simulink model "kay1024_recursive_demo"  (R2021b)
settings: Solver=FixedStepDiscrete  StartTime=0.0  StopTime=420  FixedStep=1  RelTol=1e-3
InitFcn:
  | kay_demo_init;
undefined symbols (not defined in the file or in its folder): i
libraries: hdlBasic x1189, dspsrcs4 x16, vmcUtilities x1
(part 4 of 14)

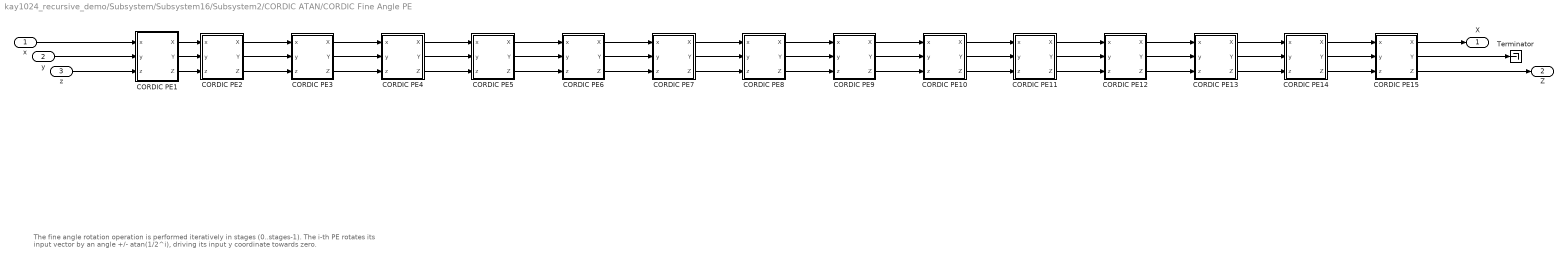
== system kay1024_recursive_demo/Subsystem/Subsystem16/Subsystem2/CORDIC ATAN/CORDIC Fine Angle PE ==
  note: The fine angle rotation operation is performed iteratively in stages (0..stages-1).
      | The i-th PE rotates its input vector by an angle +/- atan(1/2^i), driving its input y coordinate towards zero.
  x : Inport
  y : Inport  Port=2
  z : Inport  Port=3
  CORDIC PE1 : Subsystem  mask(CORDIC iteration PE){ii=0, pe_nbits=pe_nbits, pe_binpt=pe_binpt, epsilon_k_fcn=atan, epsilon_k=, pipeline=pipeline(1,1)}
      mask prompts: ii "Iteration Index ii"; pe_nbits "Number of X,Y,Z Bits"; pe_binpt "X,Y,Z Binary Point Position"; epsilon_k_fcn "Epsilon_k Function"; pipeline "Pipeline Latency"
      mask init: same as kay1024_recursive_demo/Subsystem/Subsystem16/Subsystem/CORDIC ATAN/CORDIC Fine Angle PE/CORDIC PE1
      mask TypeOptions epsilon_k_fcn: atan | atanh
      mask Display:
      | patch([0 iWidth iWidth 0],[0 0 iHeight iHeight] , bg);
      | patch(logoX,logoY , fg);
      | port_label('input',1,'x');
      | port_label('input',2,'y');
      | port_label('input',3,'z');
      | port_label('output',1,'X');
      | port_label('output',2,'Y');
      | port_label('output',3,'Z');
      | plot([0 0 iWidth iWidth 0], [0 iHeight iHeight 0 0]);
  CORDIC PE10 : Subsystem  mask(CORDIC iteration PE){ii=9, pe_nbits=pe_nbits, pe_binpt=pe_binpt, epsilon_k_fcn=atan, epsilon_k=, pipeline=pipeline(1,10)}
      mask prompts: ii "Iteration Index ii"; pe_nbits "Number of X,Y,Z Bits"; pe_binpt "X,Y,Z Binary Point Position"; epsilon_k_fcn "Epsilon_k Function"; pipeline "Pipeline Latency"
      mask init: same as kay1024_recursive_demo/Subsystem/Subsystem16/Subsystem/CORDIC ATAN/CORDIC Fine Angle PE/CORDIC PE1
      mask TypeOptions epsilon_k_fcn: atan | atanh
      mask Display:
      | patch([0 iWidth iWidth 0],[0 0 iHeight iHeight] , bg);
      | patch(logoX,logoY , fg);
      | port_label('input',1,'x');
      | port_label('input',2,'y');
      | port_label('input',3,'z');
      | port_label('output',1,'X');
      | port_label('output',2,'Y');
      | port_label('output',3,'Z');
      | plot([0 0 iWidth iWidth 0], [0 iHeight iHeight 0 0]);
  CORDIC PE11 : Subsystem  mask(CORDIC iteration PE){ii=10, pe_nbits=pe_nbits, pe_binpt=pe_binpt, epsilon_k_fcn=atan, epsilon_k=, pipeline=pipeline(1,11)}
      mask prompts: ii "Iteration Index ii"; pe_nbits "Number of X,Y,Z Bits"; pe_binpt "X,Y,Z Binary Point Position"; epsilon_k_fcn "Epsilon_k Function"; pipeline "Pipeline Latency"
      mask init: same as kay1024_recursive_demo/Subsystem/Subsystem16/Subsystem/CORDIC ATAN/CORDIC Fine Angle PE/CORDIC PE1
      mask TypeOptions epsilon_k_fcn: atan | atanh
      mask Display:
      | patch([0 iWidth iWidth 0],[0 0 iHeight iHeight] , bg);
      | patch(logoX,logoY , fg);
      | port_label('input',1,'x');
      | port_label('input',2,'y');
      | port_label('input',3,'z');
      | port_label('output',1,'X');
      | port_label('output',2,'Y');
      | port_label('output',3,'Z');
      | plot([0 0 iWidth iWidth 0], [0 iHeight iHeight 0 0]);
  CORDIC PE12 : Subsystem  mask(CORDIC iteration PE){ii=11, pe_nbits=pe_nbits, pe_binpt=pe_binpt, epsilon_k_fcn=atan, epsilon_k=, pipeline=pipeline(1,12)}
      mask prompts: ii "Iteration Index ii"; pe_nbits "Number of X,Y,Z Bits"; pe_binpt "X,Y,Z Binary Point Position"; epsilon_k_fcn "Epsilon_k Function"; pipeline "Pipeline Latency"
      mask init: same as kay1024_recursive_demo/Subsystem/Subsystem16/Subsystem/CORDIC ATAN/CORDIC Fine Angle PE/CORDIC PE1
      mask TypeOptions epsilon_k_fcn: atan | atanh
      mask Display:
      | patch([0 iWidth iWidth 0],[0 0 iHeight iHeight] , bg);
      | patch(logoX,logoY , fg);
      | port_label('input',1,'x');
      | port_label('input',2,'y');
      | port_label('input',3,'z');
      | port_label('output',1,'X');
      | port_label('output',2,'Y');
      | port_label('output',3,'Z');
      | plot([0 0 iWidth iWidth 0], [0 iHeight iHeight 0 0]);
  CORDIC PE13 : Subsystem  mask(CORDIC iteration PE){ii=12, pe_nbits=pe_nbits, pe_binpt=pe_binpt, epsilon_k_fcn=atan, epsilon_k=, pipeline=pipeline(1,13)}
      mask prompts: ii "Iteration Index ii"; pe_nbits "Number of X,Y,Z Bits"; pe_binpt "X,Y,Z Binary Point Position"; epsilon_k_fcn "Epsilon_k Function"; pipeline "Pipeline Latency"
      mask init: same as kay1024_recursive_demo/Subsystem/Subsystem16/Subsystem/CORDIC ATAN/CORDIC Fine Angle PE/CORDIC PE1
      mask TypeOptions epsilon_k_fcn: atan | atanh
      mask Display:
      | patch([0 iWidth iWidth 0],[0 0 iHeight iHeight] , bg);
      | patch(logoX,logoY , fg);
      | port_label('input',1,'x');
      | port_label('input',2,'y');
      | port_label('input',3,'z');
      | port_label('output',1,'X');
      | port_label('output',2,'Y');
      | port_label('output',3,'Z');
      | plot([0 0 iWidth iWidth 0], [0 iHeight iHeight 0 0]);
  CORDIC PE14 : Subsystem  mask(CORDIC iteration PE){ii=13, pe_nbits=pe_nbits, pe_binpt=pe_binpt, epsilon_k_fcn=atan, epsilon_k=, pipeline=pipeline(1,14)}
      mask prompts: ii "Iteration Index ii"; pe_nbits "Number of X,Y,Z Bits"; pe_binpt "X,Y,Z Binary Point Position"; epsilon_k_fcn "Epsilon_k Function"; pipeline "Pipeline Latency"
      mask init: same as kay1024_recursive_demo/Subsystem/Subsystem16/Subsystem/CORDIC ATAN/CORDIC Fine Angle PE/CORDIC PE1
      mask TypeOptions epsilon_k_fcn: atan | atanh
      mask Display:
      | patch([0 iWidth iWidth 0],[0 0 iHeight iHeight] , bg);
      | patch(logoX,logoY , fg);
      | port_label('input',1,'x');
      | port_label('input',2,'y');
      | port_label('input',3,'z');
      | port_label('output',1,'X');
      | port_label('output',2,'Y');
      | port_label('output',3,'Z');
      | plot([0 0 iWidth iWidth 0], [0 iHeight iHeight 0 0]);
  CORDIC PE15 : Subsystem  mask(CORDIC iteration PE){ii=14, pe_nbits=pe_nbits, pe_binpt=pe_binpt, epsilon_k_fcn=atan, epsilon_k=, pipeline=pipeline(1,15)}
      mask prompts: ii "Iteration Index ii"; pe_nbits "Number of X,Y,Z Bits"; pe_binpt "X,Y,Z Binary Point Position"; epsilon_k_fcn "Epsilon_k Function"; pipeline "Pipeline Latency"
      mask init: same as kay1024_recursive_demo/Subsystem/Subsystem16/Subsystem/CORDIC ATAN/CORDIC Fine Angle PE/CORDIC PE1
      mask TypeOptions epsilon_k_fcn: atan | atanh
      mask Display:
      | patch([0 iWidth iWidth 0],[0 0 iHeight iHeight] , bg);
      | patch(logoX,logoY , fg);
      | port_label('input',1,'x');
      | port_label('input',2,'y');
      | port_label('input',3,'z');
      | port_label('output',1,'X');
      | port_label('output',2,'Y');
      | port_label('output',3,'Z');
      | plot([0 0 iWidth iWidth 0], [0 iHeight iHeight 0 0]);
  CORDIC PE2 : Subsystem  mask(CORDIC iteration PE){ii=1, pe_nbits=pe_nbits, pe_binpt=pe_binpt, epsilon_k_fcn=atan, epsilon_k=, pipeline=pipeline(1,2)}
      mask prompts: ii "Iteration Index ii"; pe_nbits "Number of X,Y,Z Bits"; pe_binpt "X,Y,Z Binary Point Position"; epsilon_k_fcn "Epsilon_k Function"; pipeline "Pipeline Latency"
      mask init: same as kay1024_recursive_demo/Subsystem/Subsystem16/Subsystem/CORDIC ATAN/CORDIC Fine Angle PE/CORDIC PE1
      mask TypeOptions epsilon_k_fcn: atan | atanh
      mask Display:
      | patch([0 iWidth iWidth 0],[0 0 iHeight iHeight] , bg);
      | patch(logoX,logoY , fg);
      | port_label('input',1,'x');
      | port_label('input',2,'y');
      | port_label('input',3,'z');
      | port_label('output',1,'X');
      | port_label('output',2,'Y');
      | port_label('output',3,'Z');
      | plot([0 0 iWidth iWidth 0], [0 iHeight iHeight 0 0]);
  CORDIC PE3 : Subsystem  mask(CORDIC iteration PE){ii=2, pe_nbits=pe_nbits, pe_binpt=pe_binpt, epsilon_k_fcn=atan, epsilon_k=, pipeline=pipeline(1,3)}
      mask prompts: ii "Iteration Index ii"; pe_nbits "Number of X,Y,Z Bits"; pe_binpt "X,Y,Z Binary Point Position"; epsilon_k_fcn "Epsilon_k Function"; pipeline "Pipeline Latency"
      mask init: same as kay1024_recursive_demo/Subsystem/Subsystem16/Subsystem/CORDIC ATAN/CORDIC Fine Angle PE/CORDIC PE1
      mask TypeOptions epsilon_k_fcn: atan | atanh
      mask Display:
      | patch([0 iWidth iWidth 0],[0 0 iHeight iHeight] , bg);
      | patch(logoX,logoY , fg);
      | port_label('input',1,'x');
      | port_label('input',2,'y');
      | port_label('input',3,'z');
      | port_label('output',1,'X');
      | port_label('output',2,'Y');
      | port_label('output',3,'Z');
      | plot([0 0 iWidth iWidth 0], [0 iHeight iHeight 0 0]);
  CORDIC PE4 : Subsystem  mask(CORDIC iteration PE){ii=3, pe_nbits=pe_nbits, pe_binpt=pe_binpt, epsilon_k_fcn=atan, epsilon_k=, pipeline=pipeline(1,4)}
      mask prompts: ii "Iteration Index ii"; pe_nbits "Number of X,Y,Z Bits"; pe_binpt "X,Y,Z Binary Point Position"; epsilon_k_fcn "Epsilon_k Function"; pipeline "Pipeline Latency"
      mask init: same as kay1024_recursive_demo/Subsystem/Subsystem16/Subsystem/CORDIC ATAN/CORDIC Fine Angle PE/CORDIC PE1
      mask TypeOptions epsilon_k_fcn: atan | atanh
      mask Display:
      | patch([0 iWidth iWidth 0],[0 0 iHeight iHeight] , bg);
      | patch(logoX,logoY , fg);
      | port_label('input',1,'x');
      | port_label('input',2,'y');
      | port_label('input',3,'z');
      | port_label('output',1,'X');
      | port_label('output',2,'Y');
      | port_label('output',3,'Z');
      | plot([0 0 iWidth iWidth 0], [0 iHeight iHeight 0 0]);
  CORDIC PE5 : Subsystem  mask(CORDIC iteration PE){ii=4, pe_nbits=pe_nbits, pe_binpt=pe_binpt, epsilon_k_fcn=atan, epsilon_k=, pipeline=pipeline(1,5)}
      mask prompts: ii "Iteration Index ii"; pe_nbits "Number of X,Y,Z Bits"; pe_binpt "X,Y,Z Binary Point Position"; epsilon_k_fcn "Epsilon_k Function"; pipeline "Pipeline Latency"
      mask init: same as kay1024_recursive_demo/Subsystem/Subsystem16/Subsystem/CORDIC ATAN/CORDIC Fine Angle PE/CORDIC PE1
      mask TypeOptions epsilon_k_fcn: atan | atanh
      mask Display:
      | patch([0 iWidth iWidth 0],[0 0 iHeight iHeight] , bg);
      | patch(logoX,logoY , fg);
      | port_label('input',1,'x');
      | port_label('input',2,'y');
      | port_label('input',3,'z');
      | port_label('output',1,'X');
      | port_label('output',2,'Y');
      | port_label('output',3,'Z');
      | plot([0 0 iWidth iWidth 0], [0 iHeight iHeight 0 0]);
  CORDIC PE6 : Subsystem  mask(CORDIC iteration PE){ii=5, pe_nbits=pe_nbits, pe_binpt=pe_binpt, epsilon_k_fcn=atan, epsilon_k=, pipeline=pipeline(1,6)}
      mask prompts: ii "Iteration Index ii"; pe_nbits "Number of X,Y,Z Bits"; pe_binpt "X,Y,Z Binary Point Position"; epsilon_k_fcn "Epsilon_k Function"; pipeline "Pipeline Latency"
      mask init: same as kay1024_recursive_demo/Subsystem/Subsystem16/Subsystem/CORDIC ATAN/CORDIC Fine Angle PE/CORDIC PE1
      mask TypeOptions epsilon_k_fcn: atan | atanh
      mask Display:
      | patch([0 iWidth iWidth 0],[0 0 iHeight iHeight] , bg);
      | patch(logoX,logoY , fg);
      | port_label('input',1,'x');
      | port_label('input',2,'y');
      | port_label('input',3,'z');
      | port_label('output',1,'X');
      | port_label('output',2,'Y');
      | port_label('output',3,'Z');
      | plot([0 0 iWidth iWidth 0], [0 iHeight iHeight 0 0]);
  CORDIC PE7 : Subsystem  mask(CORDIC iteration PE){ii=6, pe_nbits=pe_nbits, pe_binpt=pe_binpt, epsilon_k_fcn=atan, epsilon_k=, pipeline=pipeline(1,7)}
      mask prompts: ii "Iteration Index ii"; pe_nbits "Number of X,Y,Z Bits"; pe_binpt "X,Y,Z Binary Point Position"; epsilon_k_fcn "Epsilon_k Function"; pipeline "Pipeline Latency"
      mask init: same as kay1024_recursive_demo/Subsystem/Subsystem16/Subsystem/CORDIC ATAN/CORDIC Fine Angle PE/CORDIC PE1
      mask TypeOptions epsilon_k_fcn: atan | atanh
      mask Display:
      | patch([0 iWidth iWidth 0],[0 0 iHeight iHeight] , bg);
      | patch(logoX,logoY , fg);
      | port_label('input',1,'x');
      | port_label('input',2,'y');
      | port_label('input',3,'z');
      | port_label('output',1,'X');
      | port_label('output',2,'Y');
      | port_label('output',3,'Z');
      | plot([0 0 iWidth iWidth 0], [0 iHeight iHeight 0 0]);
  CORDIC PE8 : Subsystem  mask(CORDIC iteration PE){ii=7, pe_nbits=pe_nbits, pe_binpt=pe_binpt, epsilon_k_fcn=atan, epsilon_k=, pipeline=pipeline(1,8)}
      mask prompts: ii "Iteration Index ii"; pe_nbits "Number of X,Y,Z Bits"; pe_binpt "X,Y,Z Binary Point Position"; epsilon_k_fcn "Epsilon_k Function"; pipeline "Pipeline Latency"
      mask init: same as kay1024_recursive_demo/Subsystem/Subsystem16/Subsystem/CORDIC ATAN/CORDIC Fine Angle PE/CORDIC PE1
      mask TypeOptions epsilon_k_fcn: atan | atanh
      mask Display:
      | patch([0 iWidth iWidth 0],[0 0 iHeight iHeight] , bg);
      | patch(logoX,logoY , fg);
      | port_label('input',1,'x');
      | port_label('input',2,'y');
      | port_label('input',3,'z');
      | port_label('output',1,'X');
      | port_label('output',2,'Y');
      | port_label('output',3,'Z');
      | plot([0 0 iWidth iWidth 0], [0 iHeight iHeight 0 0]);
  CORDIC PE9 : Subsystem  mask(CORDIC iteration PE){ii=8, pe_nbits=pe_nbits, pe_binpt=pe_binpt, epsilon_k_fcn=atan, epsilon_k=, pipeline=pipeline(1,9)}
      mask prompts: ii "Iteration Index ii"; pe_nbits "Number of X,Y,Z Bits"; pe_binpt "X,Y,Z Binary Point Position"; epsilon_k_fcn "Epsilon_k Function"; pipeline "Pipeline Latency"
      mask init: same as kay1024_recursive_demo/Subsystem/Subsystem16/Subsystem/CORDIC ATAN/CORDIC Fine Angle PE/CORDIC PE1
      mask TypeOptions epsilon_k_fcn: atan | atanh
      mask Display:
      | patch([0 iWidth iWidth 0],[0 0 iHeight iHeight] , bg);
      | patch(logoX,logoY , fg);
      | port_label('input',1,'x');
      | port_label('input',2,'y');
      | port_label('input',3,'z');
      | port_label('output',1,'X');
      | port_label('output',2,'Y');
      | port_label('output',3,'Z');
      | plot([0 0 iWidth iWidth 0], [0 iHeight iHeight 0 0]);
  Terminator : Terminator
  X : Outport
  Z : Outport  Port=2
  wires:
  CORDIC PE1/1(X) -> CORDIC PE2/1(x)
  CORDIC PE1/2(Y) -> CORDIC PE2/2(y)
  CORDIC PE1/3(Z) -> CORDIC PE2/3(z)
  CORDIC PE2/1(X) -> CORDIC PE3/1(x)
  CORDIC PE2/2(Y) -> CORDIC PE3/2(y)
  CORDIC PE2/3(Z) -> CORDIC PE3/3(z)
  CORDIC PE3/1(X) -> CORDIC PE4/1(x)
  CORDIC PE3/2(Y) -> CORDIC PE4/2(y)
  CORDIC PE3/3(Z) -> CORDIC PE4/3(z)
  CORDIC PE4/1(X) -> CORDIC PE5/1(x)
  CORDIC PE4/2(Y) -> CORDIC PE5/2(y)
  CORDIC PE4/3(Z) -> CORDIC PE5/3(z)
  CORDIC PE5/1(X) -> CORDIC PE6/1(x)
  CORDIC PE5/2(Y) -> CORDIC PE6/2(y)
  CORDIC PE5/3(Z) -> CORDIC PE6/3(z)
  CORDIC PE6/1(X) -> CORDIC PE7/1(x)
  CORDIC PE6/2(Y) -> CORDIC PE7/2(y)
  CORDIC PE6/3(Z) -> CORDIC PE7/3(z)
  CORDIC PE7/1(X) -> CORDIC PE8/1(x)
  CORDIC PE7/2(Y) -> CORDIC PE8/2(y)
  CORDIC PE7/3(Z) -> CORDIC PE8/3(z)
  CORDIC PE8/1(X) -> CORDIC PE9/1(x)
  CORDIC PE8/2(Y) -> CORDIC PE9/2(y)
  CORDIC PE8/3(Z) -> CORDIC PE9/3(z)
  CORDIC PE9/1(X) -> CORDIC PE10/1(x)
  CORDIC PE9/2(Y) -> CORDIC PE10/2(y)
  CORDIC PE9/3(Z) -> CORDIC PE10/3(z)
  CORDIC PE10/1(X) -> CORDIC PE11/1(x)
  CORDIC PE10/2(Y) -> CORDIC PE11/2(y)
  CORDIC PE10/3(Z) -> CORDIC PE11/3(z)
  CORDIC PE11/1(X) -> CORDIC PE12/1(x)
  CORDIC PE11/2(Y) -> CORDIC PE12/2(y)
  CORDIC PE11/3(Z) -> CORDIC PE12/3(z)
  CORDIC PE12/1(X) -> CORDIC PE13/1(x)
  CORDIC PE12/2(Y) -> CORDIC PE13/2(y)
  CORDIC PE12/3(Z) -> CORDIC PE13/3(z)
  CORDIC PE13/1(X) -> CORDIC PE14/1(x)
  CORDIC PE13/2(Y) -> CORDIC PE14/2(y)
  CORDIC PE13/3(Z) -> CORDIC PE14/3(z)
  CORDIC PE14/1(X) -> CORDIC PE15/1(x)
  CORDIC PE14/2(Y) -> CORDIC PE15/2(y)
  CORDIC PE14/3(Z) -> CORDIC PE15/3(z)
  x/1 -> CORDIC PE1/1(x)
  y/1 -> CORDIC PE1/2(y)
  z/1 -> CORDIC PE1/3(z)
  CORDIC PE15/1(X) -> X/1
  CORDIC PE15/2(Y) -> Terminator/1
  CORDIC PE15/3(Z) -> Z/1

== system kay1024_recursive_demo/Subsystem/Subsystem16/Subsystem2/CORDIC ATAN/Quadrant Correct ==
  note: The  CORDIC algorithm coverges for angles between  -pi/2 to +pi/2. The Quadrant Correct subsystem reflects
      | the angle back to the 2nd and 3rd quadrant from the 1st and 4th quadarnt if reflection was applied during the
      | quadarnt map stage. Reflection is applied by subtracting the output angle by pi if the original vector was in the
      | 2nd quadrant and -p if it was in the 3rd quadrant.
  Z IN : Inport
  PI_ addsub : Inport  Port=2
  Z MUX SEL : Inport  Port=3
  +PI : hdlBasic/Constant  const=pi  gui_display_data_type=Fixed-point  arith_type=Signed (2's comp)  n_bits=pe_nbits  bin_pt=pe_binpt  preci_type=Single  exp_width=8  frac_width=24  explicit_period=off  period=1  XmcBlockStatus=1  maskContainerNames=tabcontainer1  block_type=constant  block_config=sysgen:Constant_config
  -PI : hdlBasic/Constant  const=-pi  gui_display_data_type=Fixed-point  arith_type=Signed (2's comp)  n_bits=pe_nbits  bin_pt=pe_binpt  preci_type=Single  exp_width=8  frac_width=24  explicit_period=off  period=1  XmcBlockStatus=1  maskContainerNames=tabcontainer1  block_type=constant  block_config=sysgen:Constant_config
  AddSub : hdlBasic/AddSub  mode=Subtraction  use_carryin=off  use_carryout=off  en=off  latency=0  precision=User Defined  arith_type="Signed  (2's comp)"  n_bits=pe_nbits  bin_pt=pe_binpt  quantization=Truncate  overflow=Wrap  use_behavioral_HDL=on  hw_selection=Fabric  pipelined=off  use_rpm=off  XmcBlockStatus=1  maskContainerNames=tabcontainer1  block_type=addsub  block_config=sysgen:Addsub_config
  Convert : hdlBasic/Convert  gui_display_data_type=Boolean  arith_type=Boolean  n_bits=8  bin_pt=6  float_type=Single  exp_bits=8  fraction_bits=24  quantization=Truncate  overflow=Wrap  en=off  latency=0  pipeline=off  XmcBlockStatus=1  maskContainerNames=group2  block_type=convert  block_config=sysgen:Convert_config  block_width=595  block_height=885
  Mux : hdlBasic/Mux  inputs=2  en=off  latency=1  precision=Full  arith_type="Signed  (2's comp)"  n_bits=8  bin_pt=2  quantization=Truncate  overflow=Wrap  XmcBlockStatus=1  maskContainerNames=tabcontainer1  block_type=mux  block_config=sysgen:Mux_config
      settings: infoedit=Binary points are aligned automatically.<P><P>Hardware notes: A multiplexer using tristate buffers requires fewer lookup tables but is slower.
  Mux1 : hdlBasic/Mux  inputs=2  en=off  latency=0  precision=Full  arith_type="Signed  (2's comp)"  n_bits=8  bin_pt=2  quantization=Truncate  overflow=Wrap  XmcBlockStatus=1  maskContainerNames=tabcontainer1  block_type=mux  block_config=sysgen:Mux_config
      settings: infoedit=Binary points are aligned automatically.<P><P>Hardware notes: A multiplexer using tristate buffers requires fewer lookup tables but is slower.
  Z : Outport
  wires:
  -PI/1 -> Mux1/3
  +PI/1 -> Mux1/2
  Mux1/1 -> AddSub/1
  Convert/1 -> Mux1/1
  Z IN/1 -> Mux/2, AddSub/2
  Mux/1 -> Z/1
  AddSub/1 -> Mux/3
  Z MUX SEL/1 -> Mux/1
  PI_ addsub/1 -> Convert/1

== system kay1024_recursive_demo/Subsystem/Subsystem16/Subsystem2/CORDIC ATAN/Quadrant Map ==
  note: The  CORDIC algorithm converges for angles between  -pi/2 to +pi/2. The Quadrant Map subsystem always maps the
      | absolute value for x-axis. This reflects the input vector from the 2nd and 3rd quadrant to the 1st and 4th quadrant, resp.
  x : Inport
  y : Inport  Port=2
  Delay3 : hdlBasic/Delay  rst=off  en=off  latency=2  reg_retiming=off  XmcBlockStatus=1  maskContainerNames=group1  block_type=delay  block_config=sysgen:Delay_config
  Delay4 : hdlBasic/Delay  rst=off  en=off  latency=1  reg_retiming=off  XmcBlockStatus=1  maskContainerNames=group1  block_type=delay  block_config=sysgen:Delay_config
  Mux : hdlBasic/Mux  inputs=2  en=off  latency=1  precision=User Defined  arith_type="Signed  (2's comp)"  n_bits=pe_nbits  bin_pt=pe_binpt  quantization=Truncate  overflow=Wrap  XmcBlockStatus=1  maskContainerNames=tabcontainer1  block_type=mux  block_config=sysgen:Mux_config
      settings: infoedit=Binary points are aligned automatically.<P><P>Hardware notes: A multiplexer using tristate buffers requires fewer lookup tables but is slower.
  Negate1 : hdlBasic/Negate  precision=User Defined  arith_type="Signed  (2's comp)"  n_bits=pe_nbits  bin_pt=pe_binpt  quantization=Truncate  overflow=Wrap  en=off  latency=0  XmcBlockStatus=1  maskContainerNames=tabcontainer1  block_type=negate  block_config=sysgen:Negate_config
  sgn(x) : hdlBasic/Slice  nbits=1  boolean_output=off  mode=Upper Bit Location + Width  bit1=0  base1=MSB of Input  bit0=0  base0=LSB of Input  XmcBlockStatus=1  maskContainerNames=group1  block_type=slice  block_config=sysgen:Slice_config
  sgn(y) : hdlBasic/Slice  nbits=1  boolean_output=off  mode=Upper Bit Location + Width  bit1=0  base1=MSB of Input  bit0=0  base0=LSB of Input  XmcBlockStatus=1  maskContainerNames=group1  block_type=slice  block_config=sysgen:Slice_config
  X : Outport
  Y : Outport  Port=2
  sign(y) : Outport  Port=3
  sign(x) : Outport  Port=4
  wires:
  Delay3/1 -> Y/1, sgn(y)/1
  Negate1/1 -> Mux/3
  Mux/1 -> X/1
  y/1 -> Delay3/1
  x/1 -> Delay4/1
  sgn(x)/1 -> Mux/1, sign(x)/1
  sgn(y)/1 -> sign(y)/1
  Delay4/1 -> sgn(x)/1, Negate1/1, Mux/2

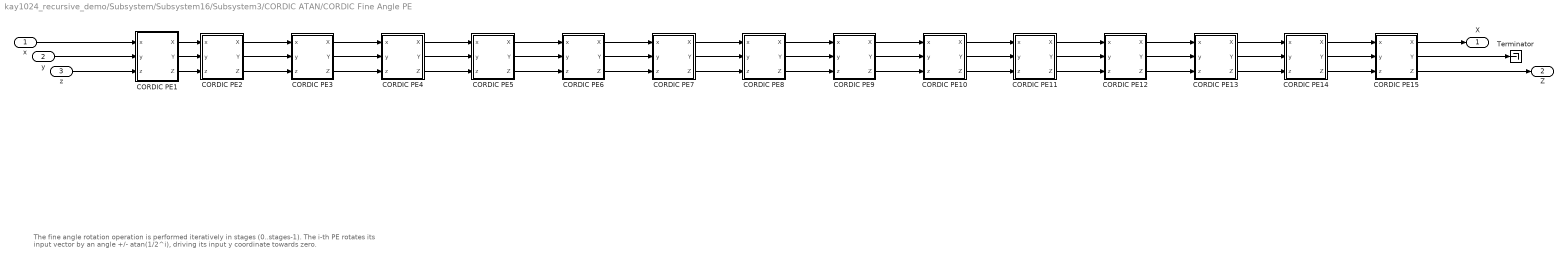
== system kay1024_recursive_demo/Subsystem/Subsystem16/Subsystem3/CORDIC ATAN/CORDIC Fine Angle PE ==
  note: The fine angle rotation operation is performed iteratively in stages (0..stages-1).
      | The i-th PE rotates its input vector by an angle +/- atan(1/2^i), driving its input y coordinate towards zero.
  x : Inport
  y : Inport  Port=2
  z : Inport  Port=3
  CORDIC PE1 : Subsystem  mask(CORDIC iteration PE){ii=0, pe_nbits=pe_nbits, pe_binpt=pe_binpt, epsilon_k_fcn=atan, epsilon_k=, pipeline=pipeline(1,1)}
      mask prompts: ii "Iteration Index ii"; pe_nbits "Number of X,Y,Z Bits"; pe_binpt "X,Y,Z Binary Point Position"; epsilon_k_fcn "Epsilon_k Function"; pipeline "Pipeline Latency"
      mask init: same as kay1024_recursive_demo/Subsystem/Subsystem16/Subsystem/CORDIC ATAN/CORDIC Fine Angle PE/CORDIC PE1
      mask TypeOptions epsilon_k_fcn: atan | atanh
      mask Display:
      | patch([0 iWidth iWidth 0],[0 0 iHeight iHeight] , bg);
      | patch(logoX,logoY , fg);
      | port_label('input',1,'x');
      | port_label('input',2,'y');
      | port_label('input',3,'z');
      | port_label('output',1,'X');
      | port_label('output',2,'Y');
      | port_label('output',3,'Z');
      | plot([0 0 iWidth iWidth 0], [0 iHeight iHeight 0 0]);
  CORDIC PE10 : Subsystem  mask(CORDIC iteration PE){ii=9, pe_nbits=pe_nbits, pe_binpt=pe_binpt, epsilon_k_fcn=atan, epsilon_k=, pipeline=pipeline(1,10)}
      mask prompts: ii "Iteration Index ii"; pe_nbits "Number of X,Y,Z Bits"; pe_binpt "X,Y,Z Binary Point Position"; epsilon_k_fcn "Epsilon_k Function"; pipeline "Pipeline Latency"
      mask init: same as kay1024_recursive_demo/Subsystem/Subsystem16/Subsystem/CORDIC ATAN/CORDIC Fine Angle PE/CORDIC PE1
      mask TypeOptions epsilon_k_fcn: atan | atanh
      mask Display:
      | patch([0 iWidth iWidth 0],[0 0 iHeight iHeight] , bg);
      | patch(logoX,logoY , fg);
      | port_label('input',1,'x');
      | port_label('input',2,'y');
      | port_label('input',3,'z');
      | port_label('output',1,'X');
      | port_label('output',2,'Y');
      | port_label('output',3,'Z');
      | plot([0 0 iWidth iWidth 0], [0 iHeight iHeight 0 0]);
  CORDIC PE11 : Subsystem  mask(CORDIC iteration PE){ii=10, pe_nbits=pe_nbits, pe_binpt=pe_binpt, epsilon_k_fcn=atan, epsilon_k=, pipeline=pipeline(1,11)}
      mask prompts: ii "Iteration Index ii"; pe_nbits "Number of X,Y,Z Bits"; pe_binpt "X,Y,Z Binary Point Position"; epsilon_k_fcn "Epsilon_k Function"; pipeline "Pipeline Latency"
      mask init: same as kay1024_recursive_demo/Subsystem/Subsystem16/Subsystem/CORDIC ATAN/CORDIC Fine Angle PE/CORDIC PE1
      mask TypeOptions epsilon_k_fcn: atan | atanh
      mask Display:
      | patch([0 iWidth iWidth 0],[0 0 iHeight iHeight] , bg);
      | patch(logoX,logoY , fg);
      | port_label('input',1,'x');
      | port_label('input',2,'y');
      | port_label('input',3,'z');
      | port_label('output',1,'X');
      | port_label('output',2,'Y');
      | port_label('output',3,'Z');
      | plot([0 0 iWidth iWidth 0], [0 iHeight iHeight 0 0]);
  CORDIC PE12 : Subsystem  mask(CORDIC iteration PE){ii=11, pe_nbits=pe_nbits, pe_binpt=pe_binpt, epsilon_k_fcn=atan, epsilon_k=, pipeline=pipeline(1,12)}
      mask prompts: ii "Iteration Index ii"; pe_nbits "Number of X,Y,Z Bits"; pe_binpt "X,Y,Z Binary Point Position"; epsilon_k_fcn "Epsilon_k Function"; pipeline "Pipeline Latency"
      mask init: same as kay1024_recursive_demo/Subsystem/Subsystem16/Subsystem/CORDIC ATAN/CORDIC Fine Angle PE/CORDIC PE1
      mask TypeOptions epsilon_k_fcn: atan | atanh
      mask Display:
      | patch([0 iWidth iWidth 0],[0 0 iHeight iHeight] , bg);
      | patch(logoX,logoY , fg);
      | port_label('input',1,'x');
      | port_label('input',2,'y');
      | port_label('input',3,'z');
      | port_label('output',1,'X');
      | port_label('output',2,'Y');
      | port_label('output',3,'Z');
      | plot([0 0 iWidth iWidth 0], [0 iHeight iHeight 0 0]);
  CORDIC PE13 : Subsystem  mask(CORDIC iteration PE){ii=12, pe_nbits=pe_nbits, pe_binpt=pe_binpt, epsilon_k_fcn=atan, epsilon_k=, pipeline=pipeline(1,13)}
      mask prompts: ii "Iteration Index ii"; pe_nbits "Number of X,Y,Z Bits"; pe_binpt "X,Y,Z Binary Point Position"; epsilon_k_fcn "Epsilon_k Function"; pipeline "Pipeline Latency"
      mask init: same as kay1024_recursive_demo/Subsystem/Subsystem16/Subsystem/CORDIC ATAN/CORDIC Fine Angle PE/CORDIC PE1
      mask TypeOptions epsilon_k_fcn: atan | atanh
      mask Display:
      | patch([0 iWidth iWidth 0],[0 0 iHeight iHeight] , bg);
      | patch(logoX,logoY , fg);
      | port_label('input',1,'x');
      | port_label('input',2,'y');
      | port_label('input',3,'z');
      | port_label('output',1,'X');
      | port_label('output',2,'Y');
      | port_label('output',3,'Z');
      | plot([0 0 iWidth iWidth 0], [0 iHeight iHeight 0 0]);
  CORDIC PE14 : Subsystem  mask(CORDIC iteration PE){ii=13, pe_nbits=pe_nbits, pe_binpt=pe_binpt, epsilon_k_fcn=atan, epsilon_k=, pipeline=pipeline(1,14)}
      mask prompts: ii "Iteration Index ii"; pe_nbits "Number of X,Y,Z Bits"; pe_binpt "X,Y,Z Binary Point Position"; epsilon_k_fcn "Epsilon_k Function"; pipeline "Pipeline Latency"
      mask init: same as kay1024_recursive_demo/Subsystem/Subsystem16/Subsystem/CORDIC ATAN/CORDIC Fine Angle PE/CORDIC PE1
      mask TypeOptions epsilon_k_fcn: atan | atanh
      mask Display:
      | patch([0 iWidth iWidth 0],[0 0 iHeight iHeight] , bg);
      | patch(logoX,logoY , fg);
      | port_label('input',1,'x');
      | port_label('input',2,'y');
      | port_label('input',3,'z');
      | port_label('output',1,'X');
      | port_label('output',2,'Y');
      | port_label('output',3,'Z');
      | plot([0 0 iWidth iWidth 0], [0 iHeight iHeight 0 0]);
  CORDIC PE15 : Subsystem  mask(CORDIC iteration PE){ii=14, pe_nbits=pe_nbits, pe_binpt=pe_binpt, epsilon_k_fcn=atan, epsilon_k=, pipeline=pipeline(1,15)}
      mask prompts: ii "Iteration Index ii"; pe_nbits "Number of X,Y,Z Bits"; pe_binpt "X,Y,Z Binary Point Position"; epsilon_k_fcn "Epsilon_k Function"; pipeline "Pipeline Latency"
      mask init: same as kay1024_recursive_demo/Subsystem/Subsystem16/Subsystem/CORDIC ATAN/CORDIC Fine Angle PE/CORDIC PE1
      mask TypeOptions epsilon_k_fcn: atan | atanh
      mask Display:
      | patch([0 iWidth iWidth 0],[0 0 iHeight iHeight] , bg);
      | patch(logoX,logoY , fg);
      | port_label('input',1,'x');
      | port_label('input',2,'y');
      | port_label('input',3,'z');
      | port_label('output',1,'X');
      | port_label('output',2,'Y');
      | port_label('output',3,'Z');
      | plot([0 0 iWidth iWidth 0], [0 iHeight iHeight 0 0]);
  CORDIC PE2 : Subsystem  mask(CORDIC iteration PE){ii=1, pe_nbits=pe_nbits, pe_binpt=pe_binpt, epsilon_k_fcn=atan, epsilon_k=, pipeline=pipeline(1,2)}
      mask prompts: ii "Iteration Index ii"; pe_nbits "Number of X,Y,Z Bits"; pe_binpt "X,Y,Z Binary Point Position"; epsilon_k_fcn "Epsilon_k Function"; pipeline "Pipeline Latency"
      mask init: same as kay1024_recursive_demo/Subsystem/Subsystem16/Subsystem/CORDIC ATAN/CORDIC Fine Angle PE/CORDIC PE1
      mask TypeOptions epsilon_k_fcn: atan | atanh
      mask Display:
      | patch([0 iWidth iWidth 0],[0 0 iHeight iHeight] , bg);
      | patch(logoX,logoY , fg);
      | port_label('input',1,'x');
      | port_label('input',2,'y');
      | port_label('input',3,'z');
      | port_label('output',1,'X');
      | port_label('output',2,'Y');
      | port_label('output',3,'Z');
      | plot([0 0 iWidth iWidth 0], [0 iHeight iHeight 0 0]);
  CORDIC PE3 : Subsystem  mask(CORDIC iteration PE){ii=2, pe_nbits=pe_nbits, pe_binpt=pe_binpt, epsilon_k_fcn=atan, epsilon_k=, pipeline=pipeline(1,3)}
      mask prompts: ii "Iteration Index ii"; pe_nbits "Number of X,Y,Z Bits"; pe_binpt "X,Y,Z Binary Point Position"; epsilon_k_fcn "Epsilon_k Function"; pipeline "Pipeline Latency"
      mask init: same as kay1024_recursive_demo/Subsystem/Subsystem16/Subsystem/CORDIC ATAN/CORDIC Fine Angle PE/CORDIC PE1
      mask TypeOptions epsilon_k_fcn: atan | atanh
      mask Display:
      | patch([0 iWidth iWidth 0],[0 0 iHeight iHeight] , bg);
      | patch(logoX,logoY , fg);
      | port_label('input',1,'x');
      | port_label('input',2,'y');
      | port_label('input',3,'z');
      | port_label('output',1,'X');
      | port_label('output',2,'Y');
      | port_label('output',3,'Z');
      | plot([0 0 iWidth iWidth 0], [0 iHeight iHeight 0 0]);
  CORDIC PE4 : Subsystem  mask(CORDIC iteration PE){ii=3, pe_nbits=pe_nbits, pe_binpt=pe_binpt, epsilon_k_fcn=atan, epsilon_k=, pipeline=pipeline(1,4)}
      mask prompts: ii "Iteration Index ii"; pe_nbits "Number of X,Y,Z Bits"; pe_binpt "X,Y,Z Binary Point Position"; epsilon_k_fcn "Epsilon_k Function"; pipeline "Pipeline Latency"
      mask init: same as kay1024_recursive_demo/Subsystem/Subsystem16/Subsystem/CORDIC ATAN/CORDIC Fine Angle PE/CORDIC PE1
      mask TypeOptions epsilon_k_fcn: atan | atanh
      mask Display:
      | patch([0 iWidth iWidth 0],[0 0 iHeight iHeight] , bg);
      | patch(logoX,logoY , fg);
      | port_label('input',1,'x');
      | port_label('input',2,'y');
      | port_label('input',3,'z');
      | port_label('output',1,'X');
      | port_label('output',2,'Y');
      | port_label('output',3,'Z');
      | plot([0 0 iWidth iWidth 0], [0 iHeight iHeight 0 0]);
  CORDIC PE5 : Subsystem  mask(CORDIC iteration PE){ii=4, pe_nbits=pe_nbits, pe_binpt=pe_binpt, epsilon_k_fcn=atan, epsilon_k=, pipeline=pipeline(1,5)}
      mask prompts: ii "Iteration Index ii"; pe_nbits "Number of X,Y,Z Bits"; pe_binpt "X,Y,Z Binary Point Position"; epsilon_k_fcn "Epsilon_k Function"; pipeline "Pipeline Latency"
      mask init: same as kay1024_recursive_demo/Subsystem/Subsystem16/Subsystem/CORDIC ATAN/CORDIC Fine Angle PE/CORDIC PE1
      mask TypeOptions epsilon_k_fcn: atan | atanh
      mask Display:
      | patch([0 iWidth iWidth 0],[0 0 iHeight iHeight] , bg);
      | patch(logoX,logoY , fg);
      | port_label('input',1,'x');
      | port_label('input',2,'y');
      | port_label('input',3,'z');
      | port_label('output',1,'X');
      | port_label('output',2,'Y');
      | port_label('output',3,'Z');
      | plot([0 0 iWidth iWidth 0], [0 iHeight iHeight 0 0]);
  CORDIC PE6 : Subsystem  mask(CORDIC iteration PE){ii=5, pe_nbits=pe_nbits, pe_binpt=pe_binpt, epsilon_k_fcn=atan, epsilon_k=, pipeline=pipeline(1,6)}
      mask prompts: ii "Iteration Index ii"; pe_nbits "Number of X,Y,Z Bits"; pe_binpt "X,Y,Z Binary Point Position"; epsilon_k_fcn "Epsilon_k Function"; pipeline "Pipeline Latency"
      mask init: same as kay1024_recursive_demo/Subsystem/Subsystem16/Subsystem/CORDIC ATAN/CORDIC Fine Angle PE/CORDIC PE1
      mask TypeOptions epsilon_k_fcn: atan | atanh
      mask Display:
      | patch([0 iWidth iWidth 0],[0 0 iHeight iHeight] , bg);
      | patch(logoX,logoY , fg);
      | port_label('input',1,'x');
      | port_label('input',2,'y');
      | port_label('input',3,'z');
      | port_label('output',1,'X');
      | port_label('output',2,'Y');
      | port_label('output',3,'Z');
      | plot([0 0 iWidth iWidth 0], [0 iHeight iHeight 0 0]);
  CORDIC PE7 : Subsystem  mask(CORDIC iteration PE){ii=6, pe_nbits=pe_nbits, pe_binpt=pe_binpt, epsilon_k_fcn=atan, epsilon_k=, pipeline=pipeline(1,7)}
      mask prompts: ii "Iteration Index ii"; pe_nbits "Number of X,Y,Z Bits"; pe_binpt "X,Y,Z Binary Point Position"; epsilon_k_fcn "Epsilon_k Function"; pipeline "Pipeline Latency"
      mask init: same as kay1024_recursive_demo/Subsystem/Subsystem16/Subsystem/CORDIC ATAN/CORDIC Fine Angle PE/CORDIC PE1
      mask TypeOptions epsilon_k_fcn: atan | atanh
      mask Display:
      | patch([0 iWidth iWidth 0],[0 0 iHeight iHeight] , bg);
      | patch(logoX,logoY , fg);
      | port_label('input',1,'x');
      | port_label('input',2,'y');
      | port_label('input',3,'z');
      | port_label('output',1,'X');
      | port_label('output',2,'Y');
      | port_label('output',3,'Z');
      | plot([0 0 iWidth iWidth 0], [0 iHeight iHeight 0 0]);
  CORDIC PE8 : Subsystem  mask(CORDIC iteration PE){ii=7, pe_nbits=pe_nbits, pe_binpt=pe_binpt, epsilon_k_fcn=atan, epsilon_k=, pipeline=pipeline(1,8)}
      mask prompts: ii "Iteration Index ii"; pe_nbits "Number of X,Y,Z Bits"; pe_binpt "X,Y,Z Binary Point Position"; epsilon_k_fcn "Epsilon_k Function"; pipeline "Pipeline Latency"
      mask init: same as kay1024_recursive_demo/Subsystem/Subsystem16/Subsystem/CORDIC ATAN/CORDIC Fine Angle PE/CORDIC PE1
      mask TypeOptions epsilon_k_fcn: atan | atanh
      mask Display:
      | patch([0 iWidth iWidth 0],[0 0 iHeight iHeight] , bg);
      | patch(logoX,logoY , fg);
      | port_label('input',1,'x');
      | port_label('input',2,'y');
      | port_label('input',3,'z');
      | port_label('output',1,'X');
      | port_label('output',2,'Y');
      | port_label('output',3,'Z');
      | plot([0 0 iWidth iWidth 0], [0 iHeight iHeight 0 0]);
  CORDIC PE9 : Subsystem  mask(CORDIC iteration PE){ii=8, pe_nbits=pe_nbits, pe_binpt=pe_binpt, epsilon_k_fcn=atan, epsilon_k=, pipeline=pipeline(1,9)}
      mask prompts: ii "Iteration Index ii"; pe_nbits "Number of X,Y,Z Bits"; pe_binpt "X,Y,Z Binary Point Position"; epsilon_k_fcn "Epsilon_k Function"; pipeline "Pipeline Latency"
      mask init: same as kay1024_recursive_demo/Subsystem/Subsystem16/Subsystem/CORDIC ATAN/CORDIC Fine Angle PE/CORDIC PE1
      mask TypeOptions epsilon_k_fcn: atan | atanh
      mask Display:
      | patch([0 iWidth iWidth 0],[0 0 iHeight iHeight] , bg);
      | patch(logoX,logoY , fg);
      | port_label('input',1,'x');
      | port_label('input',2,'y');
      | port_label('input',3,'z');
      | port_label('output',1,'X');
      | port_label('output',2,'Y');
      | port_label('output',3,'Z');
      | plot([0 0 iWidth iWidth 0], [0 iHeight iHeight 0 0]);
  Terminator : Terminator
  X : Outport
  Z : Outport  Port=2
  wires:
  CORDIC PE1/1(X) -> CORDIC PE2/1(x)
  CORDIC PE1/2(Y) -> CORDIC PE2/2(y)
  CORDIC PE1/3(Z) -> CORDIC PE2/3(z)
  CORDIC PE2/1(X) -> CORDIC PE3/1(x)
  CORDIC PE2/2(Y) -> CORDIC PE3/2(y)
  CORDIC PE2/3(Z) -> CORDIC PE3/3(z)
  CORDIC PE3/1(X) -> CORDIC PE4/1(x)
  CORDIC PE3/2(Y) -> CORDIC PE4/2(y)
  CORDIC PE3/3(Z) -> CORDIC PE4/3(z)
  CORDIC PE4/1(X) -> CORDIC PE5/1(x)
  CORDIC PE4/2(Y) -> CORDIC PE5/2(y)
  CORDIC PE4/3(Z) -> CORDIC PE5/3(z)
  CORDIC PE5/1(X) -> CORDIC PE6/1(x)
  CORDIC PE5/2(Y) -> CORDIC PE6/2(y)
  CORDIC PE5/3(Z) -> CORDIC PE6/3(z)
  CORDIC PE6/1(X) -> CORDIC PE7/1(x)
  CORDIC PE6/2(Y) -> CORDIC PE7/2(y)
  CORDIC PE6/3(Z) -> CORDIC PE7/3(z)
  CORDIC PE7/1(X) -> CORDIC PE8/1(x)
  CORDIC PE7/2(Y) -> CORDIC PE8/2(y)
  CORDIC PE7/3(Z) -> CORDIC PE8/3(z)
  CORDIC PE8/1(X) -> CORDIC PE9/1(x)
  CORDIC PE8/2(Y) -> CORDIC PE9/2(y)
  CORDIC PE8/3(Z) -> CORDIC PE9/3(z)
  CORDIC PE9/1(X) -> CORDIC PE10/1(x)
  CORDIC PE9/2(Y) -> CORDIC PE10/2(y)
  CORDIC PE9/3(Z) -> CORDIC PE10/3(z)
  CORDIC PE10/1(X) -> CORDIC PE11/1(x)
  CORDIC PE10/2(Y) -> CORDIC PE11/2(y)
  CORDIC PE10/3(Z) -> CORDIC PE11/3(z)
  CORDIC PE11/1(X) -> CORDIC PE12/1(x)
  CORDIC PE11/2(Y) -> CORDIC PE12/2(y)
  CORDIC PE11/3(Z) -> CORDIC PE12/3(z)
  CORDIC PE12/1(X) -> CORDIC PE13/1(x)
  CORDIC PE12/2(Y) -> CORDIC PE13/2(y)
  CORDIC PE12/3(Z) -> CORDIC PE13/3(z)
  CORDIC PE13/1(X) -> CORDIC PE14/1(x)
  CORDIC PE13/2(Y) -> CORDIC PE14/2(y)
  CORDIC PE13/3(Z) -> CORDIC PE14/3(z)
  CORDIC PE14/1(X) -> CORDIC PE15/1(x)
  CORDIC PE14/2(Y) -> CORDIC PE15/2(y)
  CORDIC PE14/3(Z) -> CORDIC PE15/3(z)
  x/1 -> CORDIC PE1/1(x)
  y/1 -> CORDIC PE1/2(y)
  z/1 -> CORDIC PE1/3(z)
  CORDIC PE15/1(X) -> X/1
  CORDIC PE15/2(Y) -> Terminator/1
  CORDIC PE15/3(Z) -> Z/1

== system kay1024_recursive_demo/Subsystem/Subsystem16/Subsystem3/CORDIC ATAN/Quadrant Correct ==
  note: The  CORDIC algorithm coverges for angles between  -pi/2 to +pi/2. The Quadrant Correct subsystem reflects
      | the angle back to the 2nd and 3rd quadrant from the 1st and 4th quadarnt if reflection was applied during the
      | quadarnt map stage. Reflection is applied by subtracting the output angle by pi if the original vector was in the
      | 2nd quadrant and -p if it was in the 3rd quadrant.
  Z IN : Inport
  PI_ addsub : Inport  Port=2
  Z MUX SEL : Inport  Port=3
  +PI : hdlBasic/Constant  const=pi  gui_display_data_type=Fixed-point  arith_type=Signed (2's comp)  n_bits=pe_nbits  bin_pt=pe_binpt  preci_type=Single  exp_width=8  frac_width=24  explicit_period=off  period=1  XmcBlockStatus=1  maskContainerNames=tabcontainer1  block_type=constant  block_config=sysgen:Constant_config
  -PI : hdlBasic/Constant  const=-pi  gui_display_data_type=Fixed-point  arith_type=Signed (2's comp)  n_bits=pe_nbits  bin_pt=pe_binpt  preci_type=Single  exp_width=8  frac_width=24  explicit_period=off  period=1  XmcBlockStatus=1  maskContainerNames=tabcontainer1  block_type=constant  block_config=sysgen:Constant_config
  AddSub : hdlBasic/AddSub  mode=Subtraction  use_carryin=off  use_carryout=off  en=off  latency=0  precision=User Defined  arith_type="Signed  (2's comp)"  n_bits=pe_nbits  bin_pt=pe_binpt  quantization=Truncate  overflow=Wrap  use_behavioral_HDL=on  hw_selection=Fabric  pipelined=off  use_rpm=off  XmcBlockStatus=1  maskContainerNames=tabcontainer1  block_type=addsub  block_config=sysgen:Addsub_config
  Convert : hdlBasic/Convert  gui_display_data_type=Boolean  arith_type=Boolean  n_bits=8  bin_pt=6  float_type=Single  exp_bits=8  fraction_bits=24  quantization=Truncate  overflow=Wrap  en=off  latency=0  pipeline=off  XmcBlockStatus=1  maskContainerNames=group2  block_type=convert  block_config=sysgen:Convert_config  block_width=595  block_height=885
  Mux : hdlBasic/Mux  inputs=2  en=off  latency=1  precision=Full  arith_type="Signed  (2's comp)"  n_bits=8  bin_pt=2  quantization=Truncate  overflow=Wrap  XmcBlockStatus=1  maskContainerNames=tabcontainer1  block_type=mux  block_config=sysgen:Mux_config
      settings: infoedit=Binary points are aligned automatically.<P><P>Hardware notes: A multiplexer using tristate buffers requires fewer lookup tables but is slower.
  Mux1 : hdlBasic/Mux  inputs=2  en=off  latency=0  precision=Full  arith_type="Signed  (2's comp)"  n_bits=8  bin_pt=2  quantization=Truncate  overflow=Wrap  XmcBlockStatus=1  maskContainerNames=tabcontainer1  block_type=mux  block_config=sysgen:Mux_config
      settings: infoedit=Binary points are aligned automatically.<P><P>Hardware notes: A multiplexer using tristate buffers requires fewer lookup tables but is slower.
  Z : Outport
  wires:
  -PI/1 -> Mux1/3
  +PI/1 -> Mux1/2
  Mux1/1 -> AddSub/1
  Convert/1 -> Mux1/1
  Z IN/1 -> Mux/2, AddSub/2
  Mux/1 -> Z/1
  AddSub/1 -> Mux/3
  Z MUX SEL/1 -> Mux/1
  PI_ addsub/1 -> Convert/1

== system kay1024_recursive_demo/Subsystem/Subsystem16/Subsystem3/CORDIC ATAN/Quadrant Map ==
  note: The  CORDIC algorithm converges for angles between  -pi/2 to +pi/2. The Quadrant Map subsystem always maps the
      | absolute value for x-axis. This reflects the input vector from the 2nd and 3rd quadrant to the 1st and 4th quadrant, resp.
  x : Inport
  y : Inport  Port=2
  Delay3 : hdlBasic/Delay  rst=off  en=off  latency=2  reg_retiming=off  XmcBlockStatus=1  maskContainerNames=group1  block_type=delay  block_config=sysgen:Delay_config
  Delay4 : hdlBasic/Delay  rst=off  en=off  latency=1  reg_retiming=off  XmcBlockStatus=1  maskContainerNames=group1  block_type=delay  block_config=sysgen:Delay_config
  Mux : hdlBasic/Mux  inputs=2  en=off  latency=1  precision=User Defined  arith_type="Signed  (2's comp)"  n_bits=pe_nbits  bin_pt=pe_binpt  quantization=Truncate  overflow=Wrap  XmcBlockStatus=1  maskContainerNames=tabcontainer1  block_type=mux  block_config=sysgen:Mux_config
      settings: infoedit=Binary points are aligned automatically.<P><P>Hardware notes: A multiplexer using tristate buffers requires fewer lookup tables but is slower.
  Negate1 : hdlBasic/Negate  precision=User Defined  arith_type="Signed  (2's comp)"  n_bits=pe_nbits  bin_pt=pe_binpt  quantization=Truncate  overflow=Wrap  en=off  latency=0  XmcBlockStatus=1  maskContainerNames=tabcontainer1  block_type=negate  block_config=sysgen:Negate_config
  sgn(x) : hdlBasic/Slice  nbits=1  boolean_output=off  mode=Upper Bit Location + Width  bit1=0  base1=MSB of Input  bit0=0  base0=LSB of Input  XmcBlockStatus=1  maskContainerNames=group1  block_type=slice  block_config=sysgen:Slice_config
  sgn(y) : hdlBasic/Slice  nbits=1  boolean_output=off  mode=Upper Bit Location + Width  bit1=0  base1=MSB of Input  bit0=0  base0=LSB of Input  XmcBlockStatus=1  maskContainerNames=group1  block_type=slice  block_config=sysgen:Slice_config
  X : Outport
  Y : Outport  Port=2
  sign(y) : Outport  Port=3
  sign(x) : Outport  Port=4
  wires:
  Delay3/1 -> Y/1, sgn(y)/1
  Negate1/1 -> Mux/3
  Mux/1 -> X/1
  y/1 -> Delay3/1
  x/1 -> Delay4/1
  sgn(x)/1 -> Mux/1, sign(x)/1
  sgn(y)/1 -> sign(y)/1
  Delay4/1 -> sgn(x)/1, Negate1/1, Mux/2
